simulink model "smo_rag_pskgu"  (R2012b)
settings: Solver=ode45  StartTime=0.0  StopTime=200  RelTol=1e-3
undefined symbols (not defined in the file or in its folder): des, gcbh
settings Model: Creator=Student  LastModifiedBy=Student

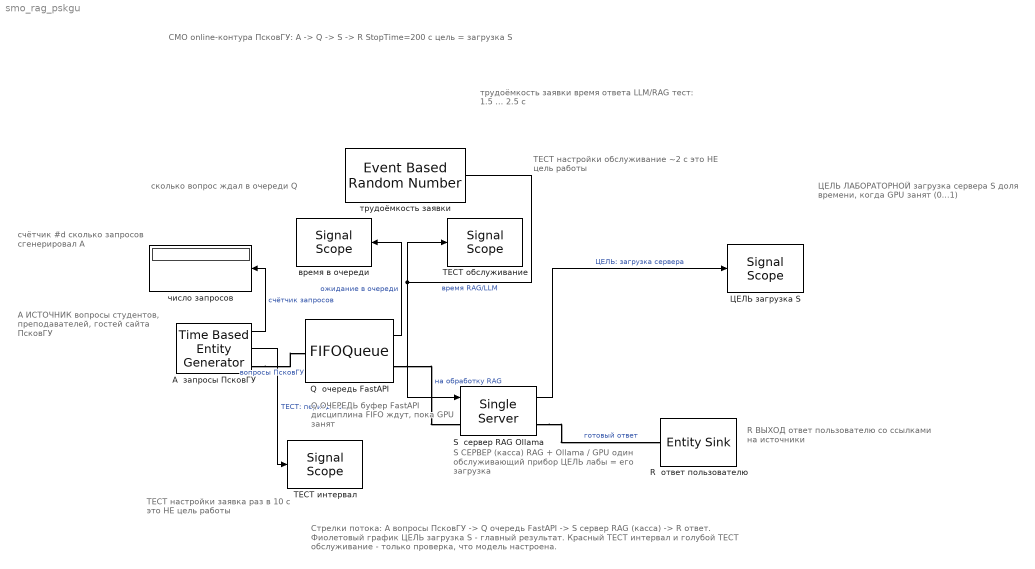
== system smo_rag_pskgu ==
  note: СМО online-контура ПсковГУ: A -> Q -> S -> R StopTime=200 с цель = загрузка S
  note: A  ИСТОЧНИК
      | вопросы студентов,
      | преподавателей, гостей
      | сайта ПсковГУ
  note: Q  ОЧЕРЕДЬ
      | буфер FastAPI
      | дисциплина FIFO
      | ждут, пока GPU занят
  note: S  СЕРВЕР (касса)
      | RAG + Ollama / GPU
      | один обслуживающий прибор
      | ЦЕЛЬ лабы = его загрузка
  note: R  ВЫХОД
      | ответ пользователю
      | со ссылками на источники
  note: трудоёмкость заявки
      | время ответа LLM/RAG
      | тест: 1.5 ... 2.5 с
  note: ТЕСТ настройки
      | заявка раз в 10 с
      | это НЕ цель работы
  note: ТЕСТ настройки
      | обслуживание ~2 с
      | это НЕ цель работы
  note: ЦЕЛЬ ЛАБОРАТОРНОЙ
      | загрузка сервера S
      | доля времени, когда
      | GPU занят (0...1)
  note: сколько вопрос
      | ждал в очереди Q
  note: счётчик #d
      | сколько запросов
      | сгенерировал A
  note: Стрелки потока:  A вопросы ПсковГУ -> Q очередь FastAPI -> S сервер RAG (касса) -> R ответ.
      | Фиолетовый график ЦЕЛЬ загрузка S - главный результат.
      | Красный ТЕСТ интервал и голубой ТЕСТ обслуживание - только проверка, что модель настроена.
  число запросов : Display
  R  ответ пользователю : EntitySink
  трудоёмкость заявки : EventBasedRandomNumber  Distribution=Uniform  meanExp=1.5  minUnif=1.5  maxUnif=2.5
  Q  очередь FastAPI : FIFOQueue  StatAverageWait=on
      settings: OutputPortMap=o2
  ТЕСТ интервал : SignalScope  LoadFcn=des.scope.CallbackSupport('seLoadFcn',gcbh)  StartFcn=des.scope.CallbackSupport('seStartFcn',gcbh)  StopFcn=des.scope.CallbackSupport('seStopFcn',gcbh)
      settings: CopyFcn=des.scope.CallbackSupport('seCopyFcn',gcbh)  DeleteFcn=des.scope.CallbackSupport('seDeleteFcn',gcbh)  PreSaveFcn=des.scope.CallbackSupport('sePreSaveFcn',gcbh)  NameChangeFcn=des.scope.CallbackSupport('seNameChangeFcn',gcbh)  OpenFcn=des.scope.CallbackSupport('seOpenFcn',gcbh)
  ТЕСТ обслуживание : SignalScope  LoadFcn=des.scope.CallbackSupport('seLoadFcn',gcbh)  StartFcn=des.scope.CallbackSupport('seStartFcn',gcbh)  StopFcn=des.scope.CallbackSupport('seStopFcn',gcbh)
      settings: CopyFcn=des.scope.CallbackSupport('seCopyFcn',gcbh)  DeleteFcn=des.scope.CallbackSupport('seDeleteFcn',gcbh)  PreSaveFcn=des.scope.CallbackSupport('sePreSaveFcn',gcbh)  NameChangeFcn=des.scope.CallbackSupport('seNameChangeFcn',gcbh)  OpenFcn=des.scope.CallbackSupport('seOpenFcn',gcbh)
  S  сервер RAG Ollama : SingleServer  ServiceTimeFrom=Signal port t  StatUtilization=on
      settings: OutputPortMap=o5
  A  запросы ПсковГУ : TimeBasedEntityGenerator  Period=10  StatNumberDeparted=on  StatAverageIntergenerationTime=on
      settings: OutputPortMap=o0,o2
  ЦЕЛЬ загрузка S : SignalScope  LoadFcn=des.scope.CallbackSupport('seLoadFcn',gcbh)  StartFcn=des.scope.CallbackSupport('seStartFcn',gcbh)  StopFcn=des.scope.CallbackSupport('seStopFcn',gcbh)
      settings: CopyFcn=des.scope.CallbackSupport('seCopyFcn',gcbh)  DeleteFcn=des.scope.CallbackSupport('seDeleteFcn',gcbh)  PreSaveFcn=des.scope.CallbackSupport('sePreSaveFcn',gcbh)  NameChangeFcn=des.scope.CallbackSupport('seNameChangeFcn',gcbh)  OpenFcn=des.scope.CallbackSupport('seOpenFcn',gcbh)
  время в очереди : SignalScope  LoadFcn=des.scope.CallbackSupport('seLoadFcn',gcbh)  StartFcn=des.scope.CallbackSupport('seStartFcn',gcbh)  StopFcn=des.scope.CallbackSupport('seStopFcn',gcbh)
      settings: CopyFcn=des.scope.CallbackSupport('seCopyFcn',gcbh)  DeleteFcn=des.scope.CallbackSupport('seDeleteFcn',gcbh)  PreSaveFcn=des.scope.CallbackSupport('sePreSaveFcn',gcbh)  NameChangeFcn=des.scope.CallbackSupport('seNameChangeFcn',gcbh)  OpenFcn=des.scope.CallbackSupport('seOpenFcn',gcbh)
  wires:
  S  сервер RAG Ollama/1 -> ЦЕЛЬ загрузка S/1  "ЦЕЛЬ: загрузка сервера"
  трудоёмкость заявки/1 -> S  сервер RAG Ollama/1, ТЕСТ обслуживание/1  "время RAG/LLM"
  A  запросы ПсковГУ/1 -> число запросов/1  "счётчик запросов"
  A  запросы ПсковГУ/2 -> ТЕСТ интервал/1  "ТЕСТ: период 10 с"
  Q  очередь FastAPI/1 -> время в очереди/1  "ожидание в очереди"
  connections:
  S  сервер RAG Ollama/RConn1 -- R  ответ пользователю/LConn1  "готовый ответ"
  Q  очередь FastAPI/RConn1 -- S  сервер RAG Ollama/LConn1  "на обработку RAG"
  A  запросы ПсковГУ/RConn1 -- Q  очередь FastAPI/LConn1  "вопросы ПсковГУ"
